simulink model "Controlador_PI"  (R2026b)
settings: Solver=VariableStepAuto
InitFcn:
  | Kp = 1.1;
  | Ki = 1.83;
settings Model: Creator=joaov  LastModifiedBy=João
settings DataIOCC: ReturnWorkspaceOutputs=off
settings ConfigComp: PLC_Enable64bitIntSupport=off  PLC_EnableStringLiteralTB=on  PLC_EnableUDTSplitting=off  PLC_EnableUnsignedAndDoubleTypes=off  PLC_FoldFBCallOutputVar=off  PLC_InlineEnumCastFunction=off  PLC_MultiTBSigbuilderTimeRange=off  PLC_RemoveUnusedSSMethodCallArguments=off  PLC_TargetIDE=codesys35  PLC_UseCallOutputArgSyntax=off

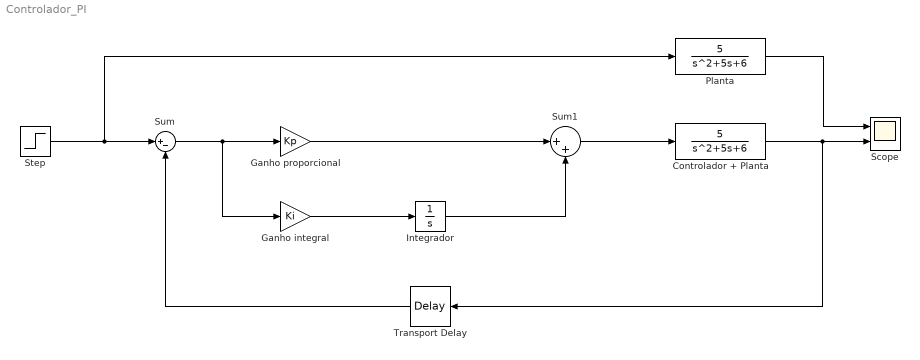
== system Controlador_PI ==
  Controlador + Planta : TransferFcn  Numerator=[5]  Denominator=[1 5 6]
  Ganho integral : Gain  Gain=Ki
  Ganho proporcional : Gain  Gain=Kp
  Integrador : Integrator
  Planta : TransferFcn  Numerator=[5]  Denominator=[1 5 6]
  Scope : Scope  NumInputPorts=2
      settings: ActiveDisplayYMinimum=17.214630716428907  ActiveDisplayYMaximum=77.665063776645738  DataLoggingVariableName=dados_continuo
  Step : Step  FinalValue=50  SampleTime=0
  Sum : Sum  Inputs=|+-
  Sum1 : Sum  Inputs=|++
  Transport Delay : TransportDelay  DelayTime=0.1
  wires:
  Controlador + Planta/1 -> Scope/2, Transport Delay/1
  Step/1 -> Planta/1, Sum/1
  Sum/1 -> Ganho integral/1, Ganho proporcional/1
  Sum1/1 -> Controlador + Planta/1
  Ganho integral/1 -> Integrador/1
  Planta/1 -> Scope/1
  Integrador/1 -> Sum1/2
  Ganho proporcional/1 -> Sum1/1
  Transport Delay/1 -> Sum/2
